simulink model "NIBB_TwoPhase_Buck"  (R2022a)
settings: Solver=VariableStepAuto  StartTime=0.0  StopTime=2  RelTol=1e-3
libraries: spsMeanLib x4, spsSeriesRLCBranchLib x4, spsDiodeLib x3, spsMosfetLib x3, spsCurrentMeasurementLib x2, eePowerMeasurement x2, spsVoltageMeasurementLib x2, spsDCVoltageSourceLib x1, spsMultimeterLib x1, spspowerguiLib x1
settings Model: Creator=Bobby  LastModifiedBy=Bobby

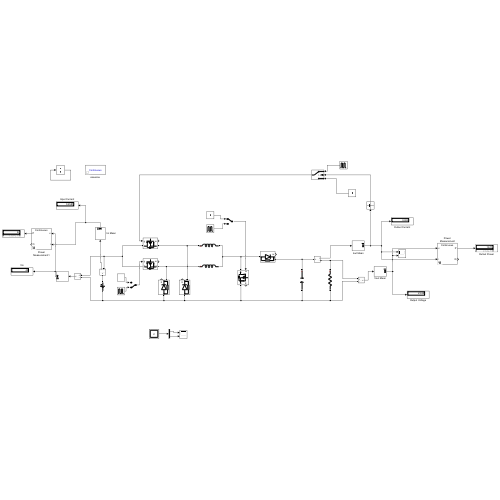
[thumbnail: Simulink's stored preview of the top-level diagram]
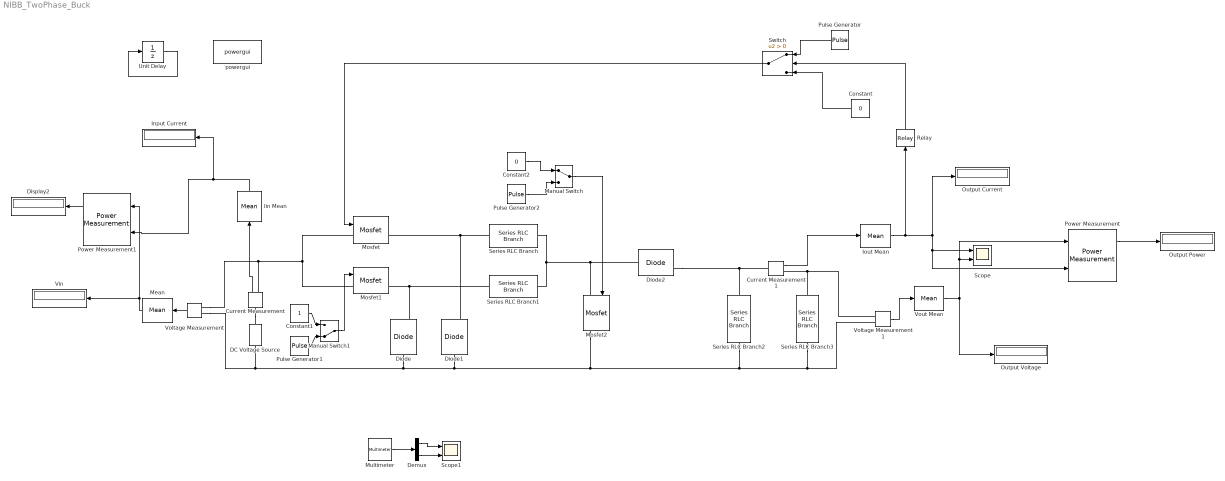
== system NIBB_TwoPhase_Buck ==
  Constant : Constant  Value=0
  Constant1 : Constant
  Constant2 : Constant  Value=0
  Current Measurement : spsCurrentMeasurementLib/Current Measurement  PhasorSimulation=off  OutputType=Complex  PSBequivalent=0
  Current Measurement1 : spsCurrentMeasurementLib/Current Measurement  PhasorSimulation=off  OutputType=Complex  PSBequivalent=0
  DC Voltage Source : spsDCVoltageSourceLib/DC Voltage Source  Amplitude=48  Measurements=None
  Demux : Demux  Outputs=2
  Diode : spsDiodeLib/Diode  Ron=0.001  Lon=0  Vf=0.8  IC=0  UseSnubber=0  Rs=500  Cs=250e-9  Measurements=on
  Diode1 : spsDiodeLib/Diode  Ron=0.001  Lon=0  Vf=0.8  IC=0  UseSnubber=0  Rs=500  Cs=250e-9  Measurements=on
  Diode2 : spsDiodeLib/Diode  Ron=0.001  Lon=0  Vf=0.8  IC=0  UseSnubber=0  Rs=500  Cs=250e-9  Measurements=on
  Display2 : Display
  Iin Mean : spsMeanLib/Mean  Freq=60  Vinit=0  Ts=0
  Input Current : Display
  Iout Mean : spsMeanLib/Mean  Freq=60  Vinit=0  Ts=0
  Manual Switch : ManualSwitch
  Manual Switch1 : ManualSwitch  CurrentSetting=0
  Mean : spsMeanLib/Mean  Freq=60  Vinit=0  Ts=0
  Mosfet : spsMosfetLib/Mosfet  Ron=0.1  Lon=0  Rd=0.01  Vfd=0  IC=0  Rs=1e5  Cs=inf  Measurements=on
  Mosfet1 : spsMosfetLib/Mosfet  Ron=0.1  Lon=0  Rd=0.01  Vfd=0  IC=0  Rs=1e5  Cs=inf  Measurements=on
  Mosfet2 : spsMosfetLib/Mosfet  Ron=0.1  Lon=0  Rd=0.01  Vfd=0  IC=0  Rs=1e5  Cs=inf  Measurements=on
  Multimeter : spsMultimeterLib/Multimeter  L=2  sel=[1 2]  yselected={}  Gain=[1 1]  OutputType=Complex  PlotAtSimulationStop=off  PhasorSimulation=off
  Output Current : Display
  Output Power : Display
  Output Voltage : Display
  Power Measurement : eePowerMeasurement/Power Measurement  LabelModeActiveChoice=Continuous  F=60  K=[0 1 2 3]  Ts=0
      settings: SourceProductBaseCode=PS
  Power Measurement1 : eePowerMeasurement/Power Measurement  LabelModeActiveChoice=Continuous  F=60  K=[0 1 2 3]  Ts=0
      settings: SourceProductBaseCode=PS
  Pulse Generator : DiscretePulseGenerator  PulseType=Time based  Period=1/50000  PulseWidth=52.3  PhaseDelay=10e-6
  Pulse Generator1 : DiscretePulseGenerator  PulseType=Time based  Period=1/50000  PulseWidth=52.3
  Pulse Generator2 : DiscretePulseGenerator  PulseType=Time based  Period=10  PulseWidth=5
  Relay : Relay  OnSwitchValue=11.5  OffSwitchValue=10.5
  Scope : Scope  NumInputPorts=2
  Scope1 : Scope  NumInputPorts=2
  Series RLC Branch : spsSeriesRLCBranchLib/Series RLC Branch  LConnTagsString=__new0  RConnTagsString=__new0  BranchType=L  Resistance=1  Inductance=80e-6  SetiL0=off  InitialCurrent=0  Capacitance=1e-6  Setx0=off  InitialVoltage=0  Measurements=Branch current
  Series RLC Branch1 : spsSeriesRLCBranchLib/Series RLC Branch  LConnTagsString=__new0  RConnTagsString=__new0  BranchType=L  Resistance=1  Inductance=80e-3  SetiL0=off  InitialCurrent=0  Capacitance=1e-6  Setx0=off  InitialVoltage=0  Measurements=Branch current
  Series RLC Branch2 : spsSeriesRLCBranchLib/Series RLC Branch  LConnTagsString=__new0  RConnTagsString=__new0  BranchType=C  Resistance=1  Inductance=1e-3  SetiL0=off  InitialCurrent=0  Capacitance=1666e-6  Setx0=off  InitialVoltage=0  Measurements=None
  Series RLC Branch3 : spsSeriesRLCBranchLib/Series RLC Branch  LConnTagsString=__new0  RConnTagsString=__new0  BranchType=R  Resistance=28.80  Inductance=1e-3  SetiL0=off  InitialCurrent=0  Capacitance=1e-6  Setx0=off  InitialVoltage=0  Measurements=None
  Switch : Switch  Criteria=u2 > Threshold  SaturateOnIntegerOverflow=off  InputSameDT=off
  Unit Delay : UnitDelay  SampleTime=-1  HasFrameUpgradeWarning=on
  Vin : Display
  Voltage Measurement : spsVoltageMeasurementLib/Voltage Measurement  PhasorSimulation=off  OutputType=Complex  PSBequivalent=0
  Voltage Measurement1 : spsVoltageMeasurementLib/Voltage Measurement  PhasorSimulation=off  OutputType=Complex  PSBequivalent=0
  Vout Mean : spsMeanLib/Mean  Freq=60  Vinit=0  Ts=0
  powergui : spspowerguiLib/powergui  Priority=1  SimulationMode=Continuous  SampleTime=50e-6  frequency=60  Iterations=50  frequencyindice=0  Pbase=100e6  ErrMax=1e-4  UnitsV=kV  UnitsW=MW  buscounter=0  FunctionMessages=off  echomessages=off  EnableUseOfTLC=off  CurrentSourceSwitches=off  DisableSnubberDevices=off  DisableRonSwitches=off  DisableVfSwitches=off  DisplayEquations=off  AutomaticDiscreteSolvers=off  SolverType=Tustin/Backward Euler (TBE)  Interpol=off  ExternalGateDelay=off  methode=off  Ts=100  x0status=blocks  SPID=on  SwTol=0  HookPort=off  NonlinearTolerance=1e-4  nMaxIteration=100  ContinueOnMaxIteration=off  RestoreLinks=warning  ResistiveCurrentMeasurement=off  Frange=[0:2:500]  Ylog=off  Xlog=on  ShowGrid=off  save=off  variable=ZData  structure=0  ZoomFFT=off  StartTime=0.0  cycles=1  DisplayStyle=1  fundamental=60  FreqAxis=off  MaxFrequency=1000  frequencyindicesteady=1  RmsSteady=1  display=off
  wires:
  Constant2/1 -> Manual Switch/1
  Pulse Generator2/1 -> Manual Switch/2
  Manual Switch/1 -> Mosfet2/1
  Constant1/1 -> Manual Switch1/1
  Pulse Generator1/1 -> Manual Switch1/2
  Manual Switch1/1 -> Mosfet1/1
  Current Measurement1/1 -> Iout Mean/1
  Voltage Measurement1/1 -> Vout Mean/1
  Iout Mean/1 -> Power Measurement/2, Scope/1, Output Current/1, Relay/1
  Vout Mean/1 -> Power Measurement/1, Scope/2, Output Voltage/1
  Power Measurement/1 -> Output Power/1
  Voltage Measurement/1 -> Mean/1
  Current Measurement/1 -> Iin Mean/1
  Mean/1 -> Vin/1, Power Measurement1/1
  Iin Mean/1 -> Input Current/1, Power Measurement1/2
  Power Measurement1/1 -> Display2/1
  Constant/1 -> Switch/3
  Relay/1 -> Switch/2
  Pulse Generator/1 -> Switch/1
  Switch/1 -> Mosfet/1
  Unit Delay/1 -> Unit Delay/1
  Multimeter/1 -> Demux/1
  Demux/2 -> Scope1/2
  Demux/1 -> Scope1/1
  connections:
  Current Measurement/LConn1 -- DC Voltage Source/RConn1
  Current Measurement/RConn1 -- Voltage Measurement/LConn1 -- Mosfet/LConn1 -- Mosfet1/LConn1
  Diode/LConn1 -- Series RLC Branch3/RConn1 -- Voltage Measurement1/LConn2 -- Series RLC Branch2/RConn1 -- Mosfet2/RConn1 -- Diode1/LConn1 -- Voltage Measurement/LConn2 -- DC Voltage Source/LConn1
  Series RLC Branch/LConn1 -- Diode1/RConn1 -- Mosfet/RConn1
  Diode/RConn1 -- Series RLC Branch1/LConn1 -- Mosfet1/RConn1
  Series RLC Branch/RConn1 -- Mosfet2/LConn1 -- Diode2/LConn1 -- Series RLC Branch1/RConn1
  Diode2/RConn1 -- Current Measurement1/LConn1 -- Series RLC Branch2/LConn1
  Series RLC Branch3/LConn1 -- Voltage Measurement1/LConn1 -- Current Measurement1/RConn1
